simulink model "ThreephaseOf_elevator_backup"  (R2025a)
settings: Solver=FixedStepDiscrete  StartTime=0.0  StopTime=16  FixedStep=5e-6  RelTol=1e-3
model workspace (MAT data in the model file):
  AFE_id_ref_profile = timeseries
  AFE_id_ref_profile.Name = 'unnamed'
  AFE_id_ref_profile.DataInfo = tsdata.datametadata
  AFE_id_ref_profile.DataInfo.Interpolation = tsdata.interpolation
  AFE_id_ref_profile.DataInfo.Interpolation.Fhandle : function handle (value not decoded)
  AFE_id_ref_profile.DataInfo.Interpolation.Name = 'linear'
  AFE_id_ref_profile.TimeInfo = tsdata.timemetadata
  AFE_id_ref_profile.TimeInfo.Length = 6
  AFE_id_ref_profile.TimeInfo.DuplicateTimes = 0
  AFE_id_ref_profile.TimeInfo.Time_ = [0; 0.1; 2; 3; 3.1; 5]
  AFE_id_ref_profile.TimeInfo.Initialized = 1
  AFE_id_ref_profile.QualityInfo = tsdata.qualmetadata
  AFE_id_ref_profile.Data_ = [0.5; 0.5; 0.5; 0.5; -0.5; -0.5]
  G = 10
  Jeq = 0.8325
  Tgravity = 27.25
  eta = 0.9
  g = 9.81
  mc = 500
  mcw = 600
  mp = 200
  r = 0.25
  speed_cmd = timeseries
  speed_cmd.Name = 'unnamed'
  speed_cmd.DataInfo = tsdata.datametadata
  speed_cmd.DataInfo.Interpolation = tsdata.interpolation
  speed_cmd.DataInfo.Interpolation.Fhandle : function handle (value not decoded)
  speed_cmd.DataInfo.Interpolation.Name = 'linear'
  speed_cmd.TimeInfo = tsdata.timemetadata
  speed_cmd.TimeInfo.Length = 6
  speed_cmd.TimeInfo.DuplicateTimes = 0
  speed_cmd.TimeInfo.Time_ = [0; 0.1; 2; 3; 3.01; 5]
  speed_cmd.TimeInfo.Initialized = 1
  speed_cmd.QualityInfo = tsdata.qualmetadata
  speed_cmd.Data_ = [0; 0; 382; 382; 0; 0]
undefined symbols (not defined in the file): DiscIntNeverNeededParam, dspblkCoreblockFVToolHelper, gcbh
libraries: simulink x6, spsSeriesRLCBranchLib x4, slpidlib x3, spsIGBTDiodeLib x3, spsThreePhaseVIMeasurementLib x3, spsBreakerLib x2, spsCurrentMeasurementLib x2, spsUniversalBridgeLib x2, eePmsmFieldOrientedControl x1, spsPermanentMagnetSynchronousMachineLib x1, spsSupercapacitorLib x1, spsThreePhaseSeriesRLCBranchLib x1
settings Model: SimulationMode=accelerator  Creator=kesav  LastModifiedBy=THIRUMALAI
settings SolverCC: ZeroCrossAlgorithm=Adaptive

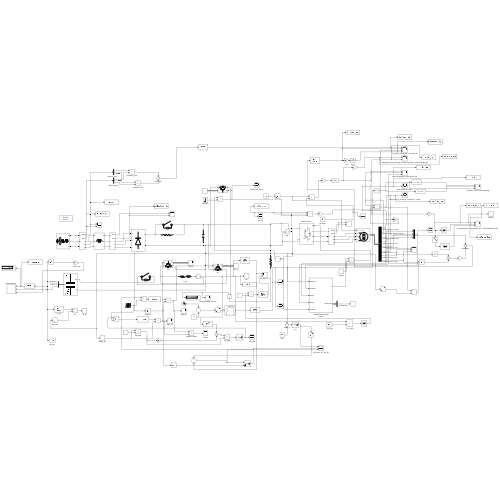
[thumbnail: Simulink's stored preview of the top-level diagram]
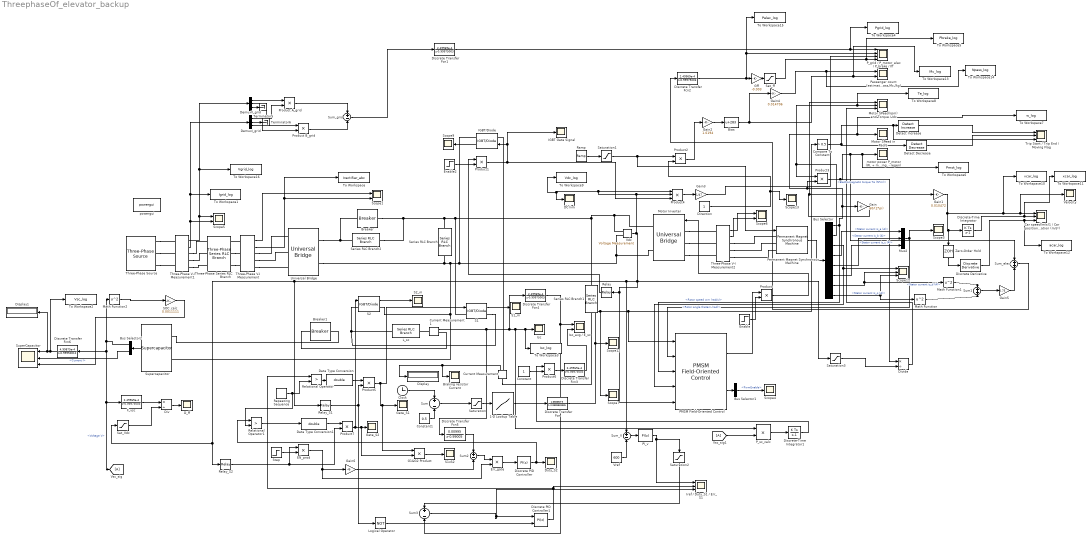
== system ThreephaseOf_elevator_backup ==
  1-D Lookup Table : Lookup_n-D  NumberOfTableDimensions=1  BreakpointsForDimension1=[0 0.2 2.25 12.2 14.25 15 ]  Table=[0 0 10 10 0 0 ]  ExtrapMethod=Clip  InternalRulePriority=Speed  RndMeth=Simplest
  Bias : Bias  Bias=283  SaturateOnIntegerOverflow=off
  Braking resistor Current : Scope
      settings: ActiveDisplayYMinimum=-0.00072485844007480883  ActiveDisplayYMaximum=0.0065237374150646536  DataLoggingVariableName=ScopeData26
  Breaker : spsBreakerLib/Breaker  InitialState=0  SwitchingTimes=[0.6]  External=off  BreakerResistance=0.01  SnubberResistance=1e6  SnubberCapacitance=inf  Measurements=None  MoreParameters=on  NoBreakLoop=off
  Breaker1 : spsBreakerLib/Breaker  InitialState=0  SwitchingTimes=[1]  External=off  BreakerResistance=0.01  SnubberResistance=1e6  SnubberCapacitance=inf  Measurements=None  MoreParameters=on  NoBreakLoop=off
  Bus Selector : BusSelector  OutputSignals=Rotor speed wm (rad/s),Electromagnetic torque Te (N*m),Rotor angle thetam (rad),Stator current is_a (A),Stator current is_b (A),Stator current is_c (A),Stator current is_d (A),Stator current is_q (A)
  Bus Selector1 : BusSelector  OutputSignals=PwmEnable
  Bus Selector2 : BusSelector  OutputSignals=Voltage V,Current I
  Car speed(m/s)1 / Car position (m) / Car acceleration (m/s²) : Scope  NumInputPorts=3
      settings: ActiveDisplayYMinimum=-0.13428641252648682  ActiveDisplayYMaximum=1.1341871365237706  DataLoggingVariableName=ScopeData27
  Clock : Clock
  Compare To Constant : simulink/Logic and Bit Operations/Compare To Constant  relop=>  const=0.5  OutDataTypeStr=boolean
  Constant : Constant
  Constant1 : Constant  Value=0.5
  Current Measurement : spsCurrentMeasurementLib/Current Measurement  PhasorSimulation=off  OutputType=Complex  PSBequivalent=0
  Current Measurement1 : spsCurrentMeasurementLib/Current Measurement  PhasorSimulation=off  OutputType=Complex  PSBequivalent=0
  DC link : Scope
      settings: ActiveDisplayYMinimum=-72.4843837819312  ActiveDisplayYMaximum=652.3606008831556  DataLoggingVariableName=ScopeData4
  D_ff : Scope
      settings: DataLoggingVariableName=ScopeData30
  Data Type Conversion : DataTypeConversion  OutDataTypeStr=double  SaturateOnIntegerOverflow=off  RndMeth=Floor
  Data Type Conversion1 : DataTypeConversion  OutDataTypeStr=double  SaturateOnIntegerOverflow=off  RndMeth=Floor
  DemuxI_grid : Demux  Outputs=3
  "DemuxV_grid\t" : Demux  Outputs=3
  Detect Decrease : simulink/Logic and Bit Operations/Detect Decrease  vinit=0  OutDataTypeStr=boolean
  Detect Increase : simulink/Logic and Bit Operations/Detect Increase  vinit=0  OutDataTypeStr=boolean
  Direction : Constant
  Discrete Transfer Fcn : DiscreteTransferFcn  LoadFcn=dspblkCoreblockFVToolHelper(gcbh,'load');  Numerator=[1.66665e-5]  Denominator=[1 -0.9999833335]
      settings: CopyFcn=dspblkCoreblockFVToolHelper(gcbh,'copy');  DeleteFcn=dspblkCoreblockFVToolHelper(gcbh,'close');  ModelCloseFcn=dspblkCoreblockFVToolHelper(gcbh,'close');  PreSaveFcn=dspblkCoreblockFVToolHelper(gcbh,'presave');  PostSaveFcn=dspblkCoreblockFVToolHelper(gcbh,'postsave');  CloseFcn=dspblkCoreblockFVToolHelper(gcbh,'close');
  Discrete Transfer Fcn{1..4} (4 alike) : DiscreteTransferFcn  LoadFcn=dspblkCoreblockFVToolHelper(gcbh,'load');  Numerator=[2.49969e-4]  Denominator=[1 -0.99975003]
      settings: CopyFcn=dspblkCoreblockFVToolHelper(gcbh,'copy');  DeleteFcn=dspblkCoreblockFVToolHelper(gcbh,'close');  ModelCloseFcn=dspblkCoreblockFVToolHelper(gcbh,'close');  PreSaveFcn=dspblkCoreblockFVToolHelper(gcbh,'presave');  PostSaveFcn=dspblkCoreblockFVToolHelper(gcbh,'postsave');  CloseFcn=dspblkCoreblockFVToolHelper(gcbh,'close');
  Discrete Transfer Fcn5 : DiscreteTransferFcn  LoadFcn=dspblkCoreblockFVToolHelper(gcbh,'load');  Numerator=[0.00995]  Denominator=[1 -0.99005]
      settings: CopyFcn=dspblkCoreblockFVToolHelper(gcbh,'copy');  DeleteFcn=dspblkCoreblockFVToolHelper(gcbh,'close');  ModelCloseFcn=dspblkCoreblockFVToolHelper(gcbh,'close');  PreSaveFcn=dspblkCoreblockFVToolHelper(gcbh,'presave');  PostSaveFcn=dspblkCoreblockFVToolHelper(gcbh,'postsave');  CloseFcn=dspblkCoreblockFVToolHelper(gcbh,'close');
  Discrete Transfer Fcn6 : DiscreteTransferFcn  LoadFcn=dspblkCoreblockFVToolHelper(gcbh,'load');  Numerator=[4.99875e-4]  Denominator=[1 -0.99950012]
      settings: CopyFcn=dspblkCoreblockFVToolHelper(gcbh,'copy');  DeleteFcn=dspblkCoreblockFVToolHelper(gcbh,'close');  ModelCloseFcn=dspblkCoreblockFVToolHelper(gcbh,'close');  PreSaveFcn=dspblkCoreblockFVToolHelper(gcbh,'presave');  PostSaveFcn=dspblkCoreblockFVToolHelper(gcbh,'postsave');  CloseFcn=dspblkCoreblockFVToolHelper(gcbh,'close');
  Discrete Derivative : simulink/Discrete/Discrete Derivative  gainval=1  ICPrevScaledInput=0  OutMin=[]  OutMax=[]  OutDataType=fixdt(1, 16)  OutScaling=2^-10  DoSatur=off
  Discrete PID Controller : slpidlib/PID Controller  Controller=PI  Form=Parallel  TimeDomain=Discrete-time  UseExternalTs=off  SampleTime=-1  IntegratorMethod=Forward Euler  FilterMethod=Forward Euler  ControllerParametersSource=internal  P=0.002  I=0.5  UseKiTs=off  D=0  UseExternalDerivativeSource=off  N=100  UseFilter=on  TunerSelectOption=Transfer Function Based (PID Tuner App)  InitialConditionSource=internal  InitialConditionForIntegrator=0.35  InitialConditionForFilter=0  DifferentiatorICPrevScaledInput=0  ExternalReset=none  TrackingMode=off  Kt=1  LimitOutput=on  SatLimitsSource=internal  UpperSaturationLimit=0.70  LowerSaturationLimit=0  LinearizeAsGain=off  AntiWindupMode=clamping  Kb=1  LimitIntegrator=off  UpperIntegratorSaturationLimit=inf  LowerIntegratorSaturationLimit=-inf  POutMin=[]  POutMax=[]  IOutMin=[]  IOutMax=[]  DOutMin=[]  DOutMax=[]  NOutMin=[]  NOutMax=[]  SumOutMin=[]  SumOutMax=[]  SaturationOutMin=[]  SaturationOutMax=[]  PParamMin=[]  PParamMax=[]  IParamMin=[]  IParamMax=[]  DParamMin=[]  DParamMax=[]  NParamMin=[]  NParamMax=[]  KbParamMin=[]  KbParamMax=[]  KtParamMin=[]  KtParamMax=[]  KbOutMin=[]  KbOutMax=[]  KtOutMin=[]  KtOutMax=[]  IntegratorOutMin=[]  IntegratorOutMax=[]  FilterOutMin=[]  FilterOutMax=[]  SumI1OutMin=[]  SumI1OutMax=[]  SumI2OutMin=[]  SumI2OutMax=[]  SumI3OutMin=[]  SumI3OutMax=[]  SumI4OutMin=[]  SumI4OutMax=[]  SumDOutMin=[]  SumDOutMax=[]  DifferentiatorOutMin=[]  DifferentiatorOutMax=[]  FilterDiffOutCoefMin=[]  FilterDiffOutCoefMax=[]  ReciprocalOutMin=[]  ReciprocalOutMax=[]  SumDenOutMin=[]  SumDenOutMax=[]  SumNumOutMin=[]  SumNumOutMax=[]  DivideOutMin=[]  DivideOutMax=[]  UdiffTsProdOutMin=[]  UdiffTsProdOutMax=[]  NTsProdOutMin=[]  NTsProdOutMax=[]  UintegralTsProdOutMin=[]  UintegralTsProdOutMax=[]  UngainTsProdOutMin=[]  UngainTsProdOutMax=[]  ClampingZeroOutDataTypeStr=Inherit: Inherit via back propagation  ClampingZeroOutMin=[]  ClampingZeroOutMax=[]  FilterDenConstantOutDataTypeStr=Inherit: Inherit via back propagation  FilterDenConstantOutMin=[]  FilterDenConstantOutMax=[]  PCopyOutDataTypeStr=Inherit: Inherit via back propagation  PCopyOutMin=[]  PCopyOutMax=[]  NCopyOutDataTypeStr=Inherit: Inherit via back propagation  NCopyOutMin=[]  NCopyOutMax=[]  IntegratorContinuousStateAttributes=''  IntegratorStateMustResolveToSignalObject=off  IntegratorRTWStateStorageClass=Auto  FilterContinuousStateAttributes=''  FilterStateMustResolveToSignalObject=off  FilterRTWStateStorageClass=Auto  ParallelPVariant=InternalParameters  IdealPVariant=Disabled  IVariant=InternalParameters  DVariant=Disabled  IntegratorVariant=Discrete  SatVariant=Enabled  AWVariant=DiscClampingParallel  PCopyVariant=Disabled  TRVariant=Disabled  FdbkBlocksVariant=Forward  IdealPFdbkVariant=Disabled  SatFdbkVariant=Disabled  DerivativeFilterVariant=Disabled  NVariant=Disabled  NCopyVariant=Disabled_SignalSpec  FilterICVariant=Disabled  IntegratorICVariant=InternalICs  ExternalResetVariant=Disabled  TRSumVariant=Passthrough  SumFdbkVariant=Disabled  SumVariant=Sum_PI  TsampFilterVariant=InternalTs  TsampNgainVariant=Passthrough  TsampIntegralVariant=Disabled_SignalSpec  ExternalSaturationOutDataTypeStr=Inherit: Same as second input  DerivativeSourceVariant=Disabled  PreIntVariant=InternalPreInt
      settings: LibrarySourceBlock=simulink/Discrete/Discrete PID Controller
  Discrete PID Controller1 : slpidlib/PID Controller  Controller=PI  Form=Parallel  TimeDomain=Discrete-time  UseExternalTs=off  SampleTime=-1  IntegratorMethod=Forward Euler  FilterMethod=Forward Euler  ControllerParametersSource=internal  P=0.002  I=0.5  UseKiTs=off  D=0  UseExternalDerivativeSource=off  N=100  UseFilter=on  TunerSelectOption=Transfer Function Based (PID Tuner App)  InitialConditionSource=internal  InitialConditionForIntegrator=0.35  InitialConditionForFilter=0  DifferentiatorICPrevScaledInput=0  ExternalReset=level  TrackingMode=off  Kt=1  LimitOutput=on  SatLimitsSource=internal  UpperSaturationLimit=0.55  LowerSaturationLimit=0  LinearizeAsGain=off  AntiWindupMode=clamping  Kb=1  LimitIntegrator=off  UpperIntegratorSaturationLimit=inf  LowerIntegratorSaturationLimit=-inf  POutMin=[]  POutMax=[]  IOutMin=[]  IOutMax=[]  DOutMin=[]  DOutMax=[]  NOutMin=[]  NOutMax=[]  SumOutMin=[]  SumOutMax=[]  SaturationOutMin=[]  SaturationOutMax=[]  PParamMin=[]  PParamMax=[]  IParamMin=[]  IParamMax=[]  DParamMin=[]  DParamMax=[]  NParamMin=[]  NParamMax=[]  KbParamMin=[]  KbParamMax=[]  KtParamMin=[]  KtParamMax=[]  KbOutMin=[]  KbOutMax=[]  KtOutMin=[]  KtOutMax=[]  IntegratorOutMin=[]  IntegratorOutMax=[]  FilterOutMin=[]  FilterOutMax=[]  SumI1OutMin=[]  SumI1OutMax=[]  SumI2OutMin=[]  SumI2OutMax=[]  SumI3OutMin=[]  SumI3OutMax=[]  SumI4OutMin=[]  SumI4OutMax=[]  SumDOutMin=[]  SumDOutMax=[]  DifferentiatorOutMin=[]  DifferentiatorOutMax=[]  FilterDiffOutCoefMin=[]  FilterDiffOutCoefMax=[]  ReciprocalOutMin=[]  ReciprocalOutMax=[]  SumDenOutMin=[]  SumDenOutMax=[]  SumNumOutMin=[]  SumNumOutMax=[]  DivideOutMin=[]  DivideOutMax=[]  UdiffTsProdOutMin=[]  UdiffTsProdOutMax=[]  NTsProdOutMin=[]  NTsProdOutMax=[]  UintegralTsProdOutMin=[]  UintegralTsProdOutMax=[]  UngainTsProdOutMin=[]  UngainTsProdOutMax=[]  ClampingZeroOutDataTypeStr=Inherit: Inherit via back propagation  ClampingZeroOutMin=[]  ClampingZeroOutMax=[]  FilterDenConstantOutDataTypeStr=Inherit: Inherit via back propagation  FilterDenConstantOutMin=[]  FilterDenConstantOutMax=[]  PCopyOutDataTypeStr=Inherit: Inherit via back propagation  PCopyOutMin=[]  PCopyOutMax=[]  NCopyOutDataTypeStr=Inherit: Inherit via back propagation  NCopyOutMin=[]  NCopyOutMax=[]  IntegratorContinuousStateAttributes=''  IntegratorStateMustResolveToSignalObject=off  IntegratorRTWStateStorageClass=Auto  FilterContinuousStateAttributes=''  FilterStateMustResolveToSignalObject=off  FilterRTWStateStorageClass=Auto  ParallelPVariant=InternalParameters  IdealPVariant=Disabled  IVariant=InternalParameters  DVariant=Disabled  IntegratorVariant=Discrete  SatVariant=Enabled  AWVariant=DiscClampingParallel  PCopyVariant=Disabled  TRVariant=Disabled  FdbkBlocksVariant=Forward  IdealPFdbkVariant=Disabled  SatFdbkVariant=Disabled  DerivativeFilterVariant=Disabled  NVariant=Disabled  NCopyVariant=Disabled_SignalSpec  FilterICVariant=Disabled  IntegratorICVariant=InternalICs  ExternalResetVariant=ExternalReset  TRSumVariant=Passthrough  SumFdbkVariant=Disabled  SumVariant=Sum_PI  TsampFilterVariant=InternalTs  TsampNgainVariant=Passthrough  TsampIntegralVariant=Disabled_SignalSpec  ExternalSaturationOutDataTypeStr=Inherit: Same as second input  DerivativeSourceVariant=Disabled  PreIntVariant=InternalPreInt
      settings: LibrarySourceBlock=simulink/Discrete/Discrete PID Controller
  Discrete-Time Integrator : DiscreteIntegrator  SampleTime=1e-4  ICPrevOutput=DiscIntNeverNeededParam  ICPrevScaledInput=DiscIntNeverNeededParam
  Discrete-Time Integrator1 : DiscreteIntegrator  SampleTime=-1  ICPrevOutput=DiscIntNeverNeededParam  ICPrevScaledInput=DiscIntNeverNeededParam
  Display : Display
  Display1 : Display
      settings: Decimation=199
  Div : Product  Inputs=*/
  Divide : Product  Inputs=*/
  Duty_S2 : Scope
      settings: ActiveDisplayYMinimum=0.32973915344384225  ActiveDisplayYMaximum=0.53234761900541994  DataLoggingVariableName=ScopeData22
  EN_prod : Product
  Enable : Step  Time=0.65  SampleTime=0
  Enable2 : Step  Time=0.65  SampleTime=0
  Err_gate : Product
  F_vsc : DiscreteTransferFcn  LoadFcn=dspblkCoreblockFVToolHelper(gcbh,'load');  Numerator=[2.49969e-4]  Denominator=[1 -0.99975003]
      settings: CopyFcn=dspblkCoreblockFVToolHelper(gcbh,'copy');  DeleteFcn=dspblkCoreblockFVToolHelper(gcbh,'close');  ModelCloseFcn=dspblkCoreblockFVToolHelper(gcbh,'close');  PreSaveFcn=dspblkCoreblockFVToolHelper(gcbh,'presave');  PostSaveFcn=dspblkCoreblockFVToolHelper(gcbh,'postsave');  CloseFcn=dspblkCoreblockFVToolHelper(gcbh,'close');
  G1&G2 Product : Product
  Gain : Gain  Gain=60/(2*pi)
  Gain1 : Gain  Gain=0.010472
  Gain2 : Gain  Gain=1.0194
  Gain3 : Gain  Gain=1/47
  Gain4 : Gain  Gain=0.014706
  Gain5 : Gain  Gain=0.75
  Gain6 : Gain  Gain=-6
  Gate_S1 : Scope
      settings: ActiveDisplayYMinimum=-0.12499999999999997  ActiveDisplayYMaximum=1.125  DataLoggingVariableName=ScopeData15
  Gate_S2 : Scope
      settings: ActiveDisplayYMinimum=-0.12499999999999997  ActiveDisplayYMaximum=1.125  DataLoggingVariableName=ScopeData21
  Gff : Gain  Gain=-0.003
  IGBT Gate Signal : Scope
      settings: ActiveDisplayYMinimum=-1  ActiveDisplayYMaximum=1  DataLoggingVariableName=ScopeData10
  IGBT/Diode : spsIGBTDiodeLib/IGBT//Diode  Ron=1e-3  Rs=1e5  Cs=inf  Measurements=on
  Iref / Duty_S1 / Err_S1 : Scope  NumInputPorts=3
      settings: ActiveDisplayYMinimum=-1.4299617185507776  ActiveDisplayYMaximum=12.869655466957001  DataLoggingVariableName=ScopeData29
  Isc : Scope
      settings: ActiveDisplayYMinimum=-13.1354172025549  ActiveDisplayYMaximum=19.125236598255839  DataLoggingVariableName=ScopeData14
  Isc_avg / E_sc : Scope  NumInputPorts=2
      settings: ActiveDisplayYMinimum=-5.9788548133694128  ActiveDisplayYMaximum=12.053424559961705  DataLoggingVariableName=ScopeData19
  L_sc : spsSeriesRLCBranchLib/Series RLC Branch  LConnTagsString=__new0  RConnTagsString=__new0  BranchType=RL  Resistance=1  Inductance=4e-3  SetiL0=off  InitialCurrent=0  Capacitance=1e-6  Setx0=off  InitialVoltage=0  Measurements=None
  Logical Operator : Logic  Operator=NOT  AllPortsSameDT=off  OutDataTypeStr=boolean
  Math Function : Math  Operator=square
  Math Function1 : Math  Operator=square
  Math Function2 : Math  Operator=square
  Motor Inverter : spsUniversalBridgeLib/Universal Bridge  Arms=3  SnubberResistance=1e5  SnubberCapacitance=inf  Device=IGBT / Diodes  Ron=1e-3  Lon=0  ForwardVoltages=[1.5 0.8]  ForwardVoltage=0  GTOparameters=[ 10e-6 , 20e-6 ]  IGBTparameters=[ 1e-6 , 2e-6 ]  Measurements=None  Measurements_2=None  converterType=Rectifier
  Motor SPeed in Rad/s : Scope
      settings: ActiveDisplayYMinimum=-1  ActiveDisplayYMaximum=1  DataLoggingVariableName=ScopeData8
  Motor SPeed(rpm)  and Torque / Idc : Scope  NumInputPorts=3
      settings: ActiveDisplayYMinimum=-1  ActiveDisplayYMaximum=1
  Mux2 : Mux  Inputs=3
  PI_v : slpidlib/PID Controller  Controller=PI  Form=Parallel  TimeDomain=Discrete-time  UseExternalTs=off  SampleTime=-1  IntegratorMethod=Forward Euler  FilterMethod=Forward Euler  ControllerParametersSource=internal  P=0.36  I=5.4  UseKiTs=off  D=0  UseExternalDerivativeSource=off  N=100  UseFilter=on  TunerSelectOption=Transfer Function Based (PID Tuner App)  InitialConditionSource=internal  InitialConditionForIntegrator=0  InitialConditionForFilter=0  DifferentiatorICPrevScaledInput=0  ExternalReset=none  TrackingMode=off  Kt=1  LimitOutput=on  SatLimitsSource=internal  UpperSaturationLimit=15  LowerSaturationLimit=0  LinearizeAsGain=off  AntiWindupMode=clamping  Kb=1  LimitIntegrator=off  UpperIntegratorSaturationLimit=inf  LowerIntegratorSaturationLimit=-inf  POutMin=[]  POutMax=[]  IOutMin=[]  IOutMax=[]  DOutMin=[]  DOutMax=[]  NOutMin=[]  NOutMax=[]  SumOutMin=[]  SumOutMax=[]  SaturationOutMin=[]  SaturationOutMax=[]  PParamMin=[]  PParamMax=[]  IParamMin=[]  IParamMax=[]  DParamMin=[]  DParamMax=[]  NParamMin=[]  NParamMax=[]  KbParamMin=[]  KbParamMax=[]  KtParamMin=[]  KtParamMax=[]  KbOutMin=[]  KbOutMax=[]  KtOutMin=[]  KtOutMax=[]  IntegratorOutMin=[]  IntegratorOutMax=[]  FilterOutMin=[]  FilterOutMax=[]  SumI1OutMin=[]  SumI1OutMax=[]  SumI2OutMin=[]  SumI2OutMax=[]  SumI3OutMin=[]  SumI3OutMax=[]  SumI4OutMin=[]  SumI4OutMax=[]  SumDOutMin=[]  SumDOutMax=[]  DifferentiatorOutMin=[]  DifferentiatorOutMax=[]  FilterDiffOutCoefMin=[]  FilterDiffOutCoefMax=[]  ReciprocalOutMin=[]  ReciprocalOutMax=[]  SumDenOutMin=[]  SumDenOutMax=[]  SumNumOutMin=[]  SumNumOutMax=[]  DivideOutMin=[]  DivideOutMax=[]  UdiffTsProdOutMin=[]  UdiffTsProdOutMax=[]  NTsProdOutMin=[]  NTsProdOutMax=[]  UintegralTsProdOutMin=[]  UintegralTsProdOutMax=[]  UngainTsProdOutMin=[]  UngainTsProdOutMax=[]  ClampingZeroOutDataTypeStr=Inherit: Inherit via back propagation  ClampingZeroOutMin=[]  ClampingZeroOutMax=[]  FilterDenConstantOutDataTypeStr=Inherit: Inherit via back propagation  FilterDenConstantOutMin=[]  FilterDenConstantOutMax=[]  PCopyOutDataTypeStr=Inherit: Inherit via back propagation  PCopyOutMin=[]  PCopyOutMax=[]  NCopyOutDataTypeStr=Inherit: Inherit via back propagation  NCopyOutMin=[]  NCopyOutMax=[]  IntegratorContinuousStateAttributes=''  IntegratorStateMustResolveToSignalObject=off  IntegratorRTWStateStorageClass=Auto  FilterContinuousStateAttributes=''  FilterStateMustResolveToSignalObject=off  FilterRTWStateStorageClass=Auto  ParallelPVariant=InternalParameters  IdealPVariant=Disabled  IVariant=InternalParameters  DVariant=Disabled  IntegratorVariant=Discrete  SatVariant=Enabled  AWVariant=DiscClampingParallel  PCopyVariant=Disabled  TRVariant=Disabled  FdbkBlocksVariant=Forward  IdealPFdbkVariant=Disabled  SatFdbkVariant=Disabled  DerivativeFilterVariant=Disabled  NVariant=Disabled  NCopyVariant=Disabled_SignalSpec  FilterICVariant=Disabled  IntegratorICVariant=InternalICs  ExternalResetVariant=Disabled  TRSumVariant=Passthrough  SumFdbkVariant=Disabled  SumVariant=Sum_PI  TsampFilterVariant=InternalTs  TsampNgainVariant=Passthrough  TsampIntegralVariant=Disabled_SignalSpec  ExternalSaturationOutDataTypeStr=Inherit: Same as second input  DerivativeSourceVariant=Disabled  PreIntVariant=InternalPreInt
      settings: LibrarySourceBlock=simulink/Discrete/Discrete PID Controller
  PMSM Field-Oriented Control : eePmsmFieldOrientedControl/PMSM Field-Oriented Control  winding_type=Wye-wound  CtrlMode=Velocity control  Vnom=560  Pmax=8000  Tmax=550  p=8  Vdc_on=100  Ts=5e-6  Tsc=1e-4  CtrlType=PI control  Kp_w=250  Ki_w=600  Kv_w=1  Kaw_w=50  RefType=Zero d-axis control  rpmVec=[0, 3000]  TqVec=[-100, 0, 100]  VdcVec=[300, 350]  PWMMode=SVM: space vector modulation  ModFactor=1  idMatrix=zeros(2,3,2)  iqMatrix=zeros(2,3,2)  psim=0.78  Ld=0.00024  Lq=0.00029  Rs=0.01  AxisAlignment=D-axis  Kp_id=15  Ki_id=250  Kaw_id=15  Kp_iq=250  Ki_iq=91  Kaw_iq=1  AxisPrio=Q-axis  ActZC=off  ActFF=on  ParamTypeFF=Constant parameters  LdFF=0.03  LqFF=0.03  psimFF=0.78  idVect=[-200, 0, 200]  iqVect=[-200, 0, 200]  LdMatrix=0.0002 * ones(3, 3)  LqMatrix=0.0002 * ones(3, 3)  psimMatrix=0.04 * ones(3, 3)  CPWMMode=SVM: space vector modulation  fsw=1000
      settings: LibrarySourceBlock=|
      | ee_sl_lib/PMSM Control/PMSM Field-Oriented
      | Control
  P_grid / P_motor_elec / P_brake / Iff : Scope  NumInputPorts=4
      settings: ActiveDisplayYMinimum=-552.61580975410425  ActiveDisplayYMaximum=4973.54228778694  DataLoggingVariableName=ScopeData20
  P_sc_calc : Product
  "Passenger count (estimate, number of people) / Load mass Mc (kg)" : Scope  NumInputPorts=2
      settings: ActiveDisplayYMinimum=-1  ActiveDisplayYMaximum=1  DataLoggingVariableName=ScopeData25
  Permanent Magnet Synchronous Machine : spsPermanentMagnetSynchronousMachineLib/Permanent Magnet Synchronous Machine  NbPhases=3  FluxDistribution=Sinusoidal  RotorType=Round  MechanicalLoad=Torque Tm  PresetModel=No  ShowDetailedParameters=on  MeasurementBus=off  Resistance=0.5  Inductance=8.5e-3  dqInductances=[8.5e-3,8.5e-3]  La=30e-3  MachineConstant=Flux linkage established by magnets (V.s)  Flux=0.78  VoltageCst=1131.8108  TorqueCst=9.36  Flat=120  Mechanical=[26.5 0.5 8 0]  PolePairs=4  InitialConditions=[0,0, 0,0]  InitialConditions5ph=[0 0 0 0 0 0]  RefAngle=Aligned with phase A axis (original Park)  IterativeDiscreteModel=Trapezoidal non iterative  TsBlock=-1  TsPowergui=0
  Product{,1..3,5..7} (7 alike) : Product
  Product A_grid : Product
  Product B_grid : Product
  Product4 : Product  Inputs=3
  Ramp : simulink/Sources/Ramp  slope=680  start=0.65  InitialOutput=0
  Relational Operator : RelationalOperator  Operator=>  OutDataTypeStr=boolean  RndMeth=Simplest  InputSameDT=off
  Relational Operator1 : RelationalOperator  Operator=>  OutDataTypeStr=boolean  RndMeth=Simplest  InputSameDT=off
  Relay : Relay  OnSwitchValue=650  OffSwitchValue=625
  Relay_S1 : Relay  OnSwitchValue=590  OffSwitchValue=580
  Relay_S2 : Relay  OnSwitchValue=570  OffSwitchValue=560  OnOutputValue=0  OffOutputValue=1
  Repeating Sequence : simulink/Sources/Repeating Sequence  rep_seq_t=[0 1e-4]  rep_seq_y=[0 1]
  S1 : spsIGBTDiodeLib/IGBT//Diode  Ron=1e-3  Rs=1e5  Cs=inf  Measurements=on
  S1_m : Scope
      settings: ActiveDisplayYMinimum=-72.465061272236753  ActiveDisplayYMaximum=652.18253554411729  DataLoggingVariableName=ScopeData17
  S1xS2 : Scope
      settings: ActiveDisplayYMinimum=-1  ActiveDisplayYMaximum=1  DataLoggingVariableName=ScopeData23
  S2 : spsIGBTDiodeLib/IGBT//Diode  Ron=1e-3  Rs=1e5  Cs=inf  Measurements=on
  S2_m : Scope
      settings: ActiveDisplayYMinimum=-95.376830493316078  ActiveDisplayYMaximum=691.59331944471523  DataLoggingVariableName=ScopeData28
  SOC_calc : Gain  Gain=0.0011111
  Sat_Vdc : Saturate  UpperLimit=700  LowerLimit=400
  Sat_ff : Saturate  UpperLimit=15  LowerLimit=0
  Saturation : Saturate  UpperLimit=15  LowerLimit=0
  Saturation1 : Saturate  UpperLimit=340  LowerLimit=0
  Saturation2 : Saturate  UpperLimit=15  LowerLimit=0
  Saturation3 : Saturate  UpperLimit=700  LowerLimit=300
  Scope1 : Scope  NumInputPorts=2
      settings: ActiveDisplayYMinimum=-731.89443458999938  ActiveDisplayYMaximum=731.89529007593683  DataLoggingVariableName=ScopeData7
  Scope11 : Scope  NumInputPorts=3
      settings: ActiveDisplayYMinimum=-1  ActiveDisplayYMaximum=1  DataLoggingVariableName=ScopeData11
  Scope{3..4,7,9,12..13} (6 alike) : Scope
      Scope12 settings: ActiveDisplayYMinimum=-1  ActiveDisplayYMaximum=1  DataLoggingVariableName=ScopeData12
      Scope13 settings: DataLoggingVariableName=ScopeData16
      Scope3 settings: ActiveDisplayYMinimum=-60.994771911318729  ActiveDisplayYMaximum=60.958665833551912
      Scope4 settings: ActiveDisplayYMinimum=-1  ActiveDisplayYMaximum=1  DataLoggingVariableName=ScopeData2
      Scope7 settings: ActiveDisplayYMinimum=-1  ActiveDisplayYMaximum=1  DataLoggingVariableName=ScopeData6
      Scope9 settings: ActiveDisplayYMinimum=-81.2203454839147  ActiveDisplayYMaximum=730.98310935523239  DataLoggingVariableName=ScopeData9
  Scope5 : Scope  NumInputPorts=2
      settings: ActiveDisplayYMinimum=-733.6779224669699  ActiveDisplayYMaximum=733.68515319096  DataLoggingVariableName=ScopeData3
  Scope6 : Scope  NumInputPorts=2
      settings: ActiveDisplayYMinimum=-768.54603230693237  ActiveDisplayYMaximum=768.53630731741112  DataLoggingVariableName=ScopeData5
  Series RLC Branch : spsSeriesRLCBranchLib/Series RLC Branch  LConnTagsString=__new0  RConnTagsString=__new0  BranchType=C  Resistance=0.01  Inductance=1e-3  SetiL0=off  InitialCurrent=0  Capacitance=3e-3  Setx0=on  InitialVoltage=0  Measurements=None
  Series RLC Branch1 : spsSeriesRLCBranchLib/Series RLC Branch  LConnTagsString=__new0  RConnTagsString=__new0  BranchType=R  Resistance=47  Inductance=1e-3  SetiL0=off  InitialCurrent=0  Capacitance=1e-6  Setx0=off  InitialVoltage=0  Measurements=None
  Series RLC Branch2 : spsSeriesRLCBranchLib/Series RLC Branch  LConnTagsString=__new0  RConnTagsString=__new0  BranchType=R  Resistance=50  Inductance=1e-3  SetiL0=off  InitialCurrent=0  Capacitance=1e-6  Setx0=off  InitialVoltage=0  Measurements=None
  Step : Step  Time=1e6  SampleTime=0
  Sum : Sum  Inputs=+-
  Sum1 : Sum
  Sum2 : Sum  Inputs=+-
  Sum3 : Sum  Inputs=+-
  Sum_V : Sum  Inputs=+-
  Sum_elec : Sum
  Sum_grid : Sum  Inputs=+-
  "SuperCapacitor " : Scope  NumInputPorts=3
      settings: ActiveDisplayYMinimum=286.67888391480841  ActiveDisplayYMaximum=297.71002082632123  DataLoggingVariableName=ScopeData31
  Supercapacitor : spsSupercapacitorLib/Supercapacitor  C=1.2  Rdc=0.9  Voltage=300  Ns=1  Np=1  Vinit=300  Temp=25  Nc=1  r=1e-9  epsilon=6.0208e-10  Ioc=10  Vself=[300 298.75 294.1 279.06]
      settings: LibrarySourceBlock=sps_lib/Sources/Supercapacitor
  Terminator5 : Terminator
  Terminator6 : Terminator
  Three-Phase Series RLC Branch : spsThreePhaseSeriesRLCBranchLib/Three-Phase Series RLC Branch  LConnTagsString=A|B|C  RConnTagsString=A|B|C  BranchType=L  Resistance=0.5  Inductance=5e-3  Capacitance=1e-6  Measurements=None
  Three-Phase V-I Measurement : spsThreePhaseVIMeasurementLib/Three-Phase V-I Measurement  VoltageMeasurement=phase-to-phase  SetLabelV=off  LabelV=Vabc  Vpu=off  VpuLL=off  CurrentMeasurement=yes  SetLabelI=off  LabelI=Iabc  Ipu=off  Pbase=100e6  Vbase=500e3  OutputType=Complex  PhasorSimulation=off  PSBequivalent=0
  Three-Phase V-I Measurement1 : spsThreePhaseVIMeasurementLib/Three-Phase V-I Measurement  VoltageMeasurement=phase-to-phase  SetLabelV=off  LabelV=Vabc  Vpu=off  VpuLL=off  CurrentMeasurement=yes  SetLabelI=off  LabelI=Iabc  Ipu=off  Pbase=100e6  Vbase=500e3  OutputType=Complex  PhasorSimulation=off  PSBequivalent=0
  Three-Phase V-I Measurement2 : spsThreePhaseVIMeasurementLib/Three-Phase V-I Measurement  VoltageMeasurement=phase-to-phase  SetLabelV=off  LabelV=Vabc  Vpu=off  VpuLL=off  CurrentMeasurement=yes  SetLabelI=off  LabelI=Iabc  Ipu=off  Pbase=100e6  Vbase=500e3  OutputType=Complex  PhasorSimulation=off  PSBequivalent=0
  Three-Phase Source : spsThreePhaseSourceLib/Three-Phase Source  InternalConnection=Yg  VoltagePhases=off  Voltage=415  PhaseAngle=0  Voltage_phases=[25e3 25e3 25e3]/sqrt(3)  PhaseAngles_phases=[0 -120 +120]  Frequency=50  NonIdealSource=on  SpecifyImpedance=off  Resistance=0.05  Inductance=0.5e-3  ShortCircuitLevel=100e6  BaseVoltage=25e3  XRratio=7  BusType=swing  Pref=10e3  Qref=0  Prefabc=[10e3, 10e3, 10e3]  Qrefabc=[0, 0, 0]  Qmin=-inf  Qmax=inf
  To Workspace : ToWorkspace  VariableName=Irectifier_abc  SaveFormat=Structure With Time  SampleTime=-1
  To Workspace1 : ToWorkspace  VariableName=Igrid_log  SaveFormat=Structure With Time  SampleTime=-1
  To Workspace10 : ToWorkspace  VariableName=vcar_log  SaveFormat=Timeseries  SampleTime=-1
  To Workspace11 : ToWorkspace  VariableName=xcar_log  SaveFormat=Timeseries  SampleTime=-1
  To Workspace12 : ToWorkspace  VariableName=acar_log  SaveFormat=Timeseries  SampleTime=-1
  To Workspace13 : ToWorkspace  VariableName=Mc_log  SaveFormat=Timeseries  SampleTime=-1
  To Workspace14 : ToWorkspace  VariableName=Npass_log  SaveFormat=Timeseries  SampleTime=-1
  To Workspace15 : ToWorkspace  VariableName=Pelec_log  SaveFormat=Timeseries  SampleTime=-1
  To Workspace16 : ToWorkspace  VariableName=Vgrid_log  SaveFormat=Timeseries  SampleTime=-1
  To Workspace2 : ToWorkspace  VariableName=Vsc_log  SaveFormat=Timeseries  SampleTime=-1
  To Workspace3 : ToWorkspace  VariableName=Isc_log  SaveFormat=Timeseries  SampleTime=-1
      settings: Decimation=199
  To Workspace4 : ToWorkspace  VariableName=Pgrid_log  SaveFormat=Timeseries  SampleTime=-1
      settings: Decimation=199
  To Workspace5 : ToWorkspace  VariableName=Pbrake_log  SaveFormat=Timeseries  SampleTime=-1
      settings: Decimation=199
  To Workspace6 : ToWorkspace  VariableName=Pmot_log  SaveFormat=Timeseries  SampleTime=-1
      settings: Decimation=199
  To Workspace7 : ToWorkspace  VariableName=w_log  SaveFormat=Timeseries  SampleTime=-1
  To Workspace8 : ToWorkspace  VariableName=Te_log  SaveFormat=Timeseries  SampleTime=-1
  To Workspace9 : ToWorkspace  VariableName=Vdc_log  SaveFormat=Timeseries  SampleTime=-1
  Trip Start / Trip End / Moving Flag : Scope  NumInputPorts=3
      settings: ActiveDisplayYMinimum=-1  ActiveDisplayYMaximum=1  DataLoggingVariableName=ScopeData13
  Universal Bridge : spsUniversalBridgeLib/Universal Bridge  Arms=3  SnubberResistance=1e5  SnubberCapacitance=inf  Device=Diodes  Ron=1e-3  Lon=0  ForwardVoltages="[  0  0  ]"  ForwardVoltage=0  GTOparameters=[ 10e-6 , 20e-6 ]  IGBTparameters=[ 1e-6 , 2e-6 ]  Measurements=None  Measurements_2=None  converterType=Rectifier
  Vdc : spsVoltageMeasurementLib/Voltage Measurement  PhasorSimulation=off  OutputType=Complex  PSBequivalent=0
  Velocity : Scope
      settings: ActiveDisplayYMinimum=-0.13428641252648682  ActiveDisplayYMaximum=1.1341871365237706  DataLoggingVariableName=ScopeData24
  Vref : Constant  Value=600
  Vsc_sig : Goto
  Vsc_sig1 : From
  Zero-Order Hold : ZeroOrderHold  SampleTime=1e-3
  "motor power P_motor (W, + motoring, - regen)" : Scope
      settings: ActiveDisplayYMinimum=-1  ActiveDisplayYMaximum=1  DataLoggingVariableName=ScopeData18
  powergui : sps_lib/powergui  Priority=1  SimulationMode=Discrete  SampleTime=5e-6  frequency=60  Iterations=50  frequencyindice=0  Pbase=100e6  ErrMax=1e-4  UnitsV=kV  UnitsW=MW  buscounter=0  FunctionMessages=off  echomessages=off  EnableUseOfTLC=off  CurrentSourceSwitches=off  DisableSnubberDevices=off  DisableRonSwitches=off  DisableVfSwitches=off  DisplayEquations=off  AutomaticDiscreteSolvers=off  SolverType=Tustin/Backward Euler (TBE)  Interpol=off  ExternalGateDelay=off  methode=off  Ts=100  x0status=blocks  SPID=on  SwTol=0  HookPort=off  NonlinearTolerance=1e-4  nMaxIteration=100  ContinueOnMaxIteration=off  RestoreLinks=warning  ResistiveCurrentMeasurement=off  Frange=[0:2:500]  Ylog=off  Xlog=on  ShowGrid=off  save=off  variable=ZData  structure=0  ZoomFFT=off  StartTime=0.0  cycles=1  DisplayStyle=1  fundamental=60  FreqAxis=off  MaxFrequency=1000  frequencyindicesteady=1  RmsSteady=1  display=off
  wires:
  Permanent Magnet Synchronous Machine/1 -> Bus Selector/1
  Mux2/1 -> PMSM Field-Oriented Control/2, Scope3/1
  Three-Phase V-I Measurement/2 -> To Workspace/1, Scope1/2
  Vdc/1 -> Product4/1, To Workspace9/1, DC link/1, Product4/2, Saturation3/1, PMSM Field-Oriented Control/5, Relay/1, Relay_S2/1, Sat_Vdc/1, Relay_S1/1, Sum_V/1
  PMSM Field-Oriented Control/2 -> Bus Selector1/1
  Bus Selector1/1 -> Scope4/1  "<PwmEnable>"
  Three-Phase V-I Measurement/1 -> Scope1/1
  1-D Lookup Table/1 -> Discrete Transfer Fcn/1
  Bus Selector/1 -> Gain/1, To Workspace7/1, Motor SPeed in Rad/s/1, Product3/2, PMSM Field-Oriented Control/3  "<Rotor speed wm (rad/s)>"
  Saturation1/1 -> Permanent Magnet Synchronous Machine/1, Product2/1
  Gain/1 -> Gain1/1, Motor SPeed(rpm)  and Torque / Idc/1
  Bus Selector/2 -> To Workspace8/1, Motor SPeed(rpm)  and Torque / Idc/2, Product3/1  "<Electromagnetic torque Te (N*m)>"
  Three-Phase V-I Measurement1/1 -> To Workspace16/1, "DemuxV_grid\t"/1, Scope5/1
  Three-Phase V-I Measurement1/2 -> DemuxI_grid/1, To Workspace1/1, Scope5/2
  Bus Selector/4 -> Mux2/1  "<Stator current is_a (A)>"
  Bus Selector/5 -> Mux2/2  "<Stator current is_b (A)>"
  Bus Selector/6 -> Mux2/3  "<Stator current is_c (A)>"
  Three-Phase V-I Measurement2/1 -> Scope6/1
  Three-Phase V-I Measurement2/2 -> Scope6/2
  Relay/1 -> Product1/1
  IGBT/Diode/1 -> Scope9/1
  Bus Selector/7 -> Scope11/2, Math Function1/1  "<Stator current is_d (A)>"
  Bus Selector/8 -> Scope11/3, Math Function/1  "<Stator current is_q (A)>"
  Bus Selector/3 -> PMSM Field-Oriented Control/4, Scope11/1  "<Rotor angle thetam (rad)>"
  PMSM Field-Oriented Control/1 -> Product/1
  Enable/1 -> Product/2
  Product/1 -> Motor Inverter/1
  Enable2/1 -> Product1/2
  Product1/1 -> IGBT Gate Signal/1, IGBT/Diode/1, Product4/3
  Clock/1 -> Sum/1
  Sum/1 -> Saturation/1
  Constant1/1 -> Sum/2
  Ramp/1 -> Saturation1/1
  Saturation/1 -> 1-D Lookup Table/1
  Discrete-Time Integrator/1 -> To Workspace11/1, Car speed(m/s)1 / Car position (m) / Car acceleration (m/s²)/2
  Discrete Derivative/1 -> Car speed(m/s)1 / Car position (m) / Car acceleration (m/s²)/3, To Workspace12/1
  Zero-Order Hold/1 -> Discrete Derivative/1
  Direction/1 -> Scope13/1, Product2/2
  Product2/1 -> Gain2/1
  Gain2/1 -> Bias/1
  Product3/1 -> Divide/1, "motor power P_motor (W, + motoring, - regen)"/1, To Workspace6/1, Sum_elec/1
  Product4/1 -> Gain3/1
  Gain3/1 -> P_grid / P_motor_elec / P_brake / Iff/3
  Discrete Transfer Fcn/1 -> Compare To Constant/1, PMSM Field-Oriented Control/1, Scope7/1, Scope12/1
  Detect Increase/1 -> Trip Start / Trip End / Moving Flag/1
  Detect Decrease/1 -> Trip Start / Trip End / Moving Flag/2
  Bias/1 -> Gain4/1, "Passenger count (estimate, number of people) / Load mass Mc (kg)"/2, To Workspace13/1
  Gain4/1 -> "Passenger count (estimate, number of people) / Load mass Mc (kg)"/1, To Workspace14/1
  Current Measurement/1 -> Display/1, Braking resistor Current/1
  Discrete Transfer Fcn1/1 -> To Workspace4/1, P_grid / P_motor_elec / P_brake / Iff/1
  Compare To Constant/1 -> Detect Decrease/1, Trip Start / Trip End / Moving Flag/3, Detect Increase/1
  "DemuxV_grid\t"/1 -> Product A_grid/1
  DemuxI_grid/1 -> Product A_grid/2
  "DemuxV_grid\t"/2 -> Product B_grid/1
  DemuxI_grid/3 -> Product B_grid/2
  Product A_grid/1 -> Sum_grid/1
  Product B_grid/1 -> Sum_grid/2
  "DemuxV_grid\t"/3 -> Terminator5/1
  DemuxI_grid/2 -> Terminator6/1
  Sum_grid/1 -> Discrete Transfer Fcn1/1
  Sum_elec/1 -> Discrete Transfer Fcn2/1
  Math Function1/1 -> Sum1/1
  Math Function/1 -> Sum1/2
  Sum1/1 -> Gain5/1
  Gain5/1 -> Sum_elec/2
  Product7/1 -> G1&G2 Product/2, Gate_S2/1, S2/1
  Current Measurement1/1 -> P_sc_calc/1, To Workspace3/1, Isc/1, Discrete Transfer Fcn4/1, Discrete Transfer Fcn5/1
  Repeating Sequence/1 -> Relational Operator1/2, Relational Operator/2
  Relational Operator/1 -> Data Type Conversion/1
  Data Type Conversion/1 -> Product5/1
  Relay_S1/1 -> Logical Operator/1, Product5/2
  Product5/1 -> S1/1, G1&G2 Product/1, Gate_S1/1
  S1/1 -> S1_m/1
  Discrete-Time Integrator1/1 -> Product6/1
  Constant/1 -> Product6/2
  Product6/1 -> Discrete Transfer Fcn3/1
  Discrete Transfer Fcn3/1 -> Isc_avg / E_sc/2
  Discrete Transfer Fcn4/1 -> Sum3/2, Isc_avg / E_sc/1
  Relational Operator1/1 -> Data Type Conversion1/1
  Data Type Conversion1/1 -> Product7/1
  EN_prod/1 -> Err_gate/2, Gain6/1
  Discrete Transfer Fcn5/1 -> Sum2/1
  Gain6/1 -> Sum2/2
  Discrete PID Controller/1 -> Relational Operator1/1, Duty_S2/1
  Step/1 -> EN_prod/2
  Sum2/1 -> Err_gate/1
  Err_gate/1 -> Discrete PID Controller/1
  Relay_S2/1 -> EN_prod/1, Product7/2
  G1&G2 Product/1 -> S1xS2/1
  Sum3/1 -> Iref / Duty_S1 / Err_S1/3, Discrete PID Controller1/1
  Discrete PID Controller1/1 -> Relational Operator/1, Iref / Duty_S1 / Err_S1/2
  S2/1 -> S2_m/1
  Vref/1 -> Sum_V/2
  Sum_V/1 -> PI_v/1
  PI_v/1 -> Saturation2/1, Iref / Duty_S1 / Err_S1/1
  Logical Operator/1 -> Discrete PID Controller1/2
  Gff/1 -> Sat_ff/1
  Sat_ff/1 -> To Workspace5/1, P_grid / P_motor_elec / P_brake / Iff/4
  Saturation2/1 -> Sum3/1
  Supercapacitor/1 -> Bus Selector2/1
  Bus Selector2/1 -> Vsc_sig/1, F_vsc/1, Discrete Transfer Fcn6/1, Math Function2/1  "<Voltage V>"
  Bus Selector2/2 -> "SuperCapacitor "/2  "<Current I>"
  F_vsc/1 -> Div/1
  Sat_Vdc/1 -> Div/2
  Div/1 -> D_ff/1
  Math Function2/1 -> SOC_calc/1
  SOC_calc/1 -> "SuperCapacitor "/3
  Vsc_sig1/1 -> P_sc_calc/2
  P_sc_calc/1 -> Discrete-Time Integrator1/1
  Discrete Transfer Fcn6/1 -> To Workspace2/1, Display1/1, "SuperCapacitor "/1
  Saturation3/1 -> Divide/2
  Divide/1 -> Motor SPeed(rpm)  and Torque / Idc/3
  Gain1/1 -> Zero-Order Hold/1, Discrete-Time Integrator/1, To Workspace10/1, Velocity/1, Car speed(m/s)1 / Car position (m) / Car acceleration (m/s²)/1
  Discrete Transfer Fcn2/1 -> Gff/1, P_grid / P_motor_elec / P_brake / Iff/2, To Workspace15/1
  connections:
  Three-Phase V-I Measurement/LConn1 -- Three-Phase Series RLC Branch/RConn1
  Three-Phase Series RLC Branch/RConn2 -- Three-Phase V-I Measurement/LConn2
  Three-Phase Series RLC Branch/RConn3 -- Three-Phase V-I Measurement/LConn3
  Three-Phase V-I Measurement/RConn3 -- Universal Bridge/LConn3
  Three-Phase V-I Measurement/RConn2 -- Universal Bridge/LConn2
  Three-Phase V-I Measurement/RConn1 -- Universal Bridge/LConn1
  Vdc/LConn2 -- Motor Inverter/RConn2 -- IGBT/Diode/RConn1 -- Supercapacitor/LConn2 -- S2/RConn1 -- Series RLC Branch/RConn1 -- Universal Bridge/RConn2
  Vdc/LConn1 -- Motor Inverter/RConn1 -- Series RLC Branch1/LConn1 -- S1/LConn1 -- Series RLC Branch2/RConn1 -- Breaker/RConn1 -- Series RLC Branch/LConn1
  Three-Phase Source/RConn1 -- Three-Phase V-I Measurement1/LConn1
  Three-Phase Source/RConn2 -- Three-Phase V-I Measurement1/LConn2
  Three-Phase Source/RConn3 -- Three-Phase V-I Measurement1/LConn3
  Three-Phase V-I Measurement1/RConn1 -- Three-Phase Series RLC Branch/LConn1
  Three-Phase V-I Measurement1/RConn2 -- Three-Phase Series RLC Branch/LConn2
  Three-Phase V-I Measurement1/RConn3 -- Three-Phase Series RLC Branch/LConn3
  Motor Inverter/LConn1 -- Three-Phase V-I Measurement2/LConn1
  Motor Inverter/LConn2 -- Three-Phase V-I Measurement2/LConn2
  Motor Inverter/LConn3 -- Three-Phase V-I Measurement2/LConn3
  Three-Phase V-I Measurement2/RConn1 -- Permanent Magnet Synchronous Machine/LConn1
  Three-Phase V-I Measurement2/RConn2 -- Permanent Magnet Synchronous Machine/LConn2
  Three-Phase V-I Measurement2/RConn3 -- Permanent Magnet Synchronous Machine/LConn3
  Current Measurement/LConn1 -- Series RLC Branch1/RConn1
  Universal Bridge/RConn1 -- Breaker/LConn1 -- Series RLC Branch2/LConn1
  Current Measurement/RConn1 -- IGBT/Diode/LConn1
  L_sc/LConn1 -- S2/LConn1 -- S1/RConn1
  Current Measurement1/LConn1 -- L_sc/RConn1
  Breaker1/LConn1 -- Current Measurement1/RConn1
  Supercapacitor/LConn1 -- Breaker1/RConn1
